simulink model "Full_Controller_SIM"  (R2026a)
settings: Solver=FixedStepDiscrete  StopTime=S.tspan  FixedStep=S.dt_sim  RelTol=rel_tol  AbsTol=abs_tol
StopFcn:
  | defaultToFileBlockNames(bdroot);
undefined symbols (not defined in the file): I, S
libraries: ros2lib x8
PreSaveFcn:
  | defaultToFileBlockNames(bdroot);
settings Model: DataDictionary=ros2lib.sldd  Creator=koryh  LastModifiedBy=kjhaydon
settings SimscapeCC: SimscapeNominalValues="[{\"value\":\"1\",\"unit\":\"A\"},{\"value\":\"1\",\"unit\":\"bar\"},{\"value\":\"1\",\"unit\":\"cm^2\"},{\"value\":\"1\",\"unit\":\"cm^3/s\"},{\"value\":\"1\",\"unit\":\"kJ/kg\"},{\"value\":\"1\",\"unit\":\"kW\"},{\"value\":\"1\",\"unit\":\"l\"},{\"value\":\"1\",\"unit\":\"N\"},{\"value\":\"1\",\"unit\":\"N*m\"},{\"value\":\"1\",\"unit\":\"V\"}]"  SimscapeLogType=none  SimscapeLogDataHistory=5000.0

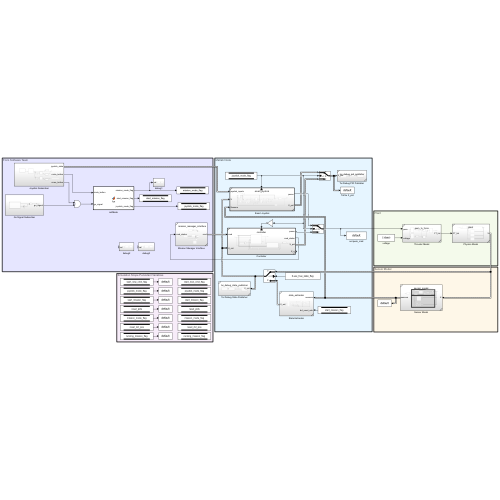
[thumbnail: Simulink's stored preview of the top-level diagram]
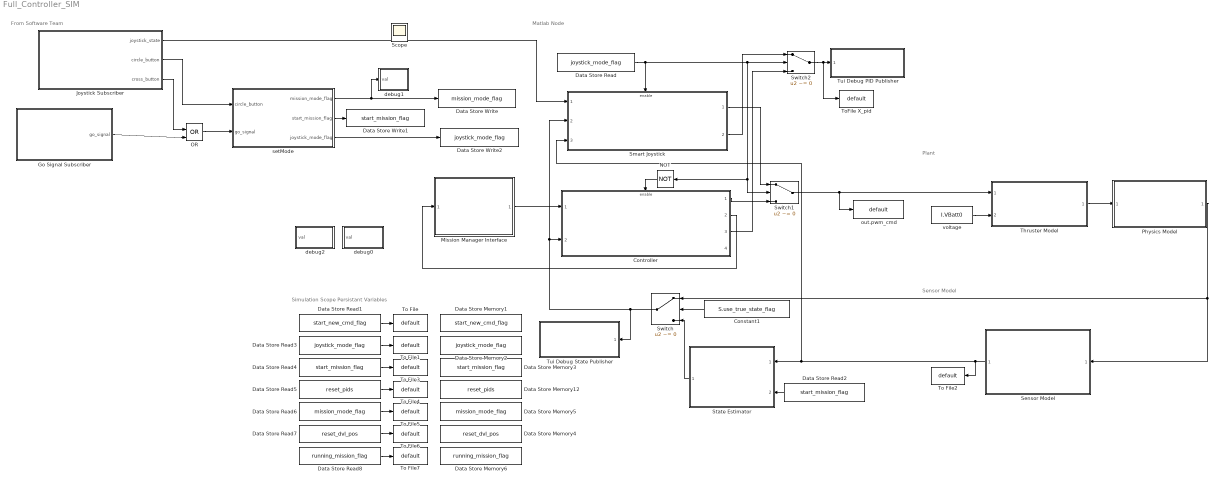
== system Full_Controller_SIM ==
  note: Sensor Model
  note: Plant
  note: Matlab Node
  note: From Software Team
  note: Simulation Scope Persistant Variables
  Constant1 : Constant  Value=S.use_true_state_flag
  Controller : Subsystem  ReferencedSubsystem=controller
  Data Store Memory1 : DataStoreMemory  DataStoreName=start_new_cmd_flag  WriteAfterWriteMsg=warning  InitialValue=true  ShowAdditionalParam=off  OutDataTypeStr=boolean
  Data Store Memory12 : DataStoreMemory  DataStoreName=reset_pids  WriteAfterWriteMsg=warning  InitialValue=false  ShowAdditionalParam=off  OutDataTypeStr=boolean
  Data Store Memory2 : DataStoreMemory  DataStoreName=joystick_mode_flag  WriteAfterWriteMsg=warning  InitialValue=S.initial_joystick_mode_enabled_flag  ShowAdditionalParam=off  OutDataTypeStr=boolean
  Data Store Memory3 : DataStoreMemory  DataStoreName=start_mission_flag  WriteAfterWriteMsg=warning  InitialValue=false  ShowAdditionalParam=off  OutDataTypeStr=boolean
  Data Store Memory4 : DataStoreMemory  DataStoreName=reset_dvl_pos  WriteAfterWriteMsg=warning  InitialValue=false  ShowAdditionalParam=off  OutDataTypeStr=boolean
  Data Store Memory5 : DataStoreMemory  DataStoreName=mission_mode_flag  WriteAfterWriteMsg=warning  InitialValue=~S.initial_joystick_mode_enabled_flag  ShowAdditionalParam=off  OutDataTypeStr=boolean
  Data Store Memory6 : DataStoreMemory  DataStoreName=running_mission_flag  WriteAfterWriteMsg=warning  InitialValue=false  ShowAdditionalParam=off  OutDataTypeStr=boolean
  Data Store Read : DataStoreRead  DataStoreName=joystick_mode_flag  IndexOptions=Index vector (dialog)  Indices=1  OutputSizes=1
  Data Store Read1 : DataStoreRead  DataStoreName=start_new_cmd_flag  IndexOptions=Index vector (dialog)  Indices=1  OutputSizes=1
  Data Store Read2 : DataStoreRead  DataStoreName=start_mission_flag  IndexOptions=Index vector (dialog)  Indices=1  OutputSizes=1
  Data Store Read3 : DataStoreRead  DataStoreName=joystick_mode_flag  IndexOptions=Index vector (dialog)  Indices=1  OutputSizes=1
  Data Store Read4 : DataStoreRead  DataStoreName=start_mission_flag  IndexOptions=Index vector (dialog)  Indices=1  OutputSizes=1
  Data Store Read5 : DataStoreRead  DataStoreName=reset_pids  IndexOptions=Index vector (dialog)  Indices=1  OutputSizes=1
  Data Store Read6 : DataStoreRead  DataStoreName=mission_mode_flag  IndexOptions=Index vector (dialog)  Indices=1  OutputSizes=1
  Data Store Read7 : DataStoreRead  DataStoreName=reset_dvl_pos  IndexOptions=Index vector (dialog)  Indices=1  OutputSizes=1
  Data Store Read8 : DataStoreRead  DataStoreName=running_mission_flag  IndexOptions=Index vector (dialog)  Indices=1  OutputSizes=1
  Data Store Write : DataStoreWrite  DataStoreName=mission_mode_flag  IndexOptions=Index vector (dialog)  Indices=1  OutputSizes=1
  Data Store Write1 : DataStoreWrite  DataStoreName=start_mission_flag  IndexOptions=Index vector (dialog)  Indices=1  OutputSizes=1
  Data Store Write2 : DataStoreWrite  DataStoreName=joystick_mode_flag  IndexOptions=Index vector (dialog)  Indices=1  OutputSizes=1
  Go Signal Subscriber : Subsystem
  Joystick Subscriber : Subsystem
  Mission Manager Interface : Subsystem  ReferencedSubsystem=mission_manager_interface
  NOT : Logic  Operator=NOT  IconShape=distinctive  AllPortsSameDT=off  OutDataTypeStr=boolean
  OR : Logic  Operator=OR  IconShape=distinctive  AllPortsSameDT=off  OutDataTypeStr=boolean
  Physics Model : Subsystem  ReferencedSubsystem=plant
  Sensor Model : Subsystem  ReferencedSubsystem=sensor_model
  Smart Joystick : Subsystem  ReferencedSubsystem=smart_joystick
  State Estimator : Subsystem  ReferencedSubsystem=state_estimator
  Switch : Switch  Criteria=u2 ~= 0  SaturateOnIntegerOverflow=off  InputSameDT=off
  Switch1 : Switch  Criteria=u2 ~= 0  SaturateOnIntegerOverflow=off  InputSameDT=off
  Switch2 : Switch  Criteria=u2 ~= 0  SaturateOnIntegerOverflow=off  InputSameDT=off
  Thruster Model : Subsystem  ReferencedSubsystem=pwm_to_force
  To File : ToFile  Filename=default  MatrixName=start_new_cmd_flag  SaveFormat=Timeseries  SampleTime=S.dt_control
  To File1 : ToFile  Filename=default  MatrixName=joystick_mode_flag  SaveFormat=Timeseries  SampleTime=S.dt_control
  To File2 : ToFile  Filename=default  MatrixName=sensors  SaveFormat=Timeseries
  To File3 : ToFile  Filename=default  MatrixName=start_mission_flag  SaveFormat=Timeseries  SampleTime=S.dt_control
  To File4 : ToFile  Filename=default  MatrixName=reset_pids  SaveFormat=Timeseries  SampleTime=S.dt_control
  To File5 : ToFile  Filename=default  MatrixName=mission_mode_flag  SaveFormat=Timeseries  SampleTime=S.dt_control
  To File6 : ToFile  Filename=default  MatrixName=reset_dvl_pos  SaveFormat=Timeseries  SampleTime=S.dt_control
  To File7 : ToFile  Filename=default  MatrixName=running_mission_flag  SaveFormat=Timeseries  SampleTime=S.dt_control
  ToFile X_pid : ToFile  Filename=default  MatrixName=X_pid  SaveFormat=Timeseries  SampleTime=S.dt_data
  Tui Debug PID Publisher : Subsystem  ReferencedSubsystem=tui_debug_pid_publisher
  Tui Debug State Publisher : Subsystem  ReferencedSubsystem=tui_debug_state_publisher
  debug0 : Subsystem
  debug1 : Subsystem
  debug2 : Subsystem
  out.pwm_cmd : ToFile  Filename=default  MatrixName=pwm_ctrl  SaveFormat=Timeseries  SampleTime=S.dt_data
  setMode : MATLAB Function  TreatAsAtomicUnit=on
  voltage : Constant  Value=I.VBatt0
  Scope : Scope
      settings: ActiveDisplayYMinimum=-0.048832566475369238  ActiveDisplayYMaximum=0.79721663606048965
  wires:
  voltage/1 -> Thruster Model/2
  Thruster Model/1 -> Physics Model/1
  Physics Model/1 -> Sensor Model/1, Switch/1
  Sensor Model/1 -> To File2/1, State Estimator/1, Smart Joystick/3
  Switch/1 -> Controller/2, Smart Joystick/2, Tui Debug State Publisher/1
  Constant1/1 -> Switch/2
  State Estimator/1 -> Switch/3
  Data Store Read2/1 -> State Estimator/2
  Controller/1 -> Switch1/3
  Switch1/1 -> out.pwm_cmd/1, Thruster Model/1
  Controller/2 -> Mission Manager Interface/1
  Go Signal Subscriber/1(go_signal) -> OR/2
  Joystick Subscriber/2(circle_button) -> setMode/1(circle_button)
  Joystick Subscriber/3(cross_button) -> OR/1
  setMode/3(joystick_mode_flag) -> Data Store Write2/1
  setMode/2(start_mission_flag) -> Data Store Write1/1
  setMode/1(mission_mode_flag) -> debug1/1(val), Data Store Write/1
  OR/1 -> setMode/2(go_signal)
  Mission Manager Interface/1 -> Controller/1
  NOT/1 -> Controller/Enable
  Data Store Read/1 -> Smart Joystick/Enable, NOT/1, Switch1/2, Switch2/2
  Smart Joystick/1 -> Switch1/1
  Joystick Subscriber/1(joystick_state) -> Smart Joystick/1
  Switch2/1 -> ToFile X_pid/1, Tui Debug PID Publisher/1
  Smart Joystick/2 -> Switch2/1
  Controller/3 -> Switch2/3
  Data Store Read3/1 -> To File1/1
  Data Store Read7/1 -> To File6/1
  Data Store Read1/1 -> To File/1
  Data Store Read5/1 -> To File4/1
  Data Store Read4/1 -> To File3/1
  Data Store Read6/1 -> To File5/1
  Data Store Read8/1 -> To File7/1

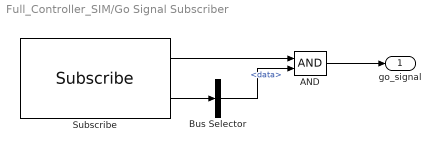
== system Full_Controller_SIM/Go Signal Subscriber ==
  AND : Logic  IconShape=distinctive  AllPortsSameDT=off  OutDataTypeStr=boolean
  Bus Selector : BusSelector  OutputSignals=data
  Subscribe : ros2lib/Subscribe  topicSource=Specify your own  topic=/go_signal  messageType=std_msgs/Bool  sampleTime=-1  QOSHistory=Keep last  QOSDepth=10  QOSReliability=Reliable  QOSDurability=Volatile  QOSDeadline=Inf  QOSLifespan=Inf  QOSLiveliness=Automatic  QOSLeaseDuration=Inf  QOSAvoidROSNamespaceConventions=off
  go_signal : Outport
  wires:
  Subscribe/2 -> Bus Selector/1
  Subscribe/1 -> AND/1
  Bus Selector/1 -> AND/2  "<data>"
  AND/1 -> go_signal/1

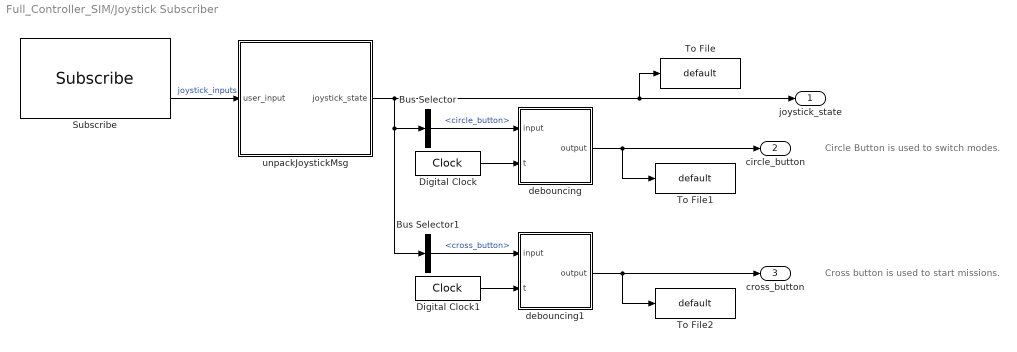
== system Full_Controller_SIM/Joystick Subscriber ==
  note: Circle Button is used to switch modes.
  note: Cross button is used to start missions.
  Bus Selector : BusSelector  OutputSignals=circle_button
  Bus Selector1 : BusSelector  OutputSignals=cross_button
  Digital Clock : DigitalClock  SampleTime=S.dt_control
  Digital Clock1 : DigitalClock  SampleTime=S.dt_control
  Subscribe : ros2lib/Subscribe  topicSource=Specify your own  topic=/ps5_controller  messageType=custom_interfaces/Gamepad  sampleTime=1/100  QOSHistory=Keep last  QOSDepth=10  QOSReliability=Reliable  QOSDurability=Volatile  QOSDeadline=Inf  QOSLifespan=Inf  QOSLiveliness=Automatic  QOSLeaseDuration=Inf  QOSAvoidROSNamespaceConventions=off
  To File : ToFile  Filename=default  MatrixName=joystick_state  SaveFormat=Timeseries  SampleTime=S.dt_control
  To File1 : ToFile  Filename=default  MatrixName=circle_button  SaveFormat=Timeseries  SampleTime=S.dt_control
  To File2 : ToFile  Filename=default  MatrixName=cross_button  SaveFormat=Timeseries  SampleTime=S.dt_control
  debouncing : MATLAB Function  TreatAsAtomicUnit=on
  debouncing1 : MATLAB Function  TreatAsAtomicUnit=on
  unpackJoystickMsg : MATLAB Function  TreatAsAtomicUnit=on
  joystick_state : Outport
  circle_button : Outport  Port=2
  cross_button : Outport  Port=3
  wires:
  Subscribe/2 -> unpackJoystickMsg/1(user_input)  "joystick_inputs"
  debouncing/1(output) -> circle_button/1, To File1/1
  Digital Clock/1 -> debouncing/2(t)
  Bus Selector/1 -> debouncing/1(input)  "<circle_button>"
  unpackJoystickMsg/1(joystick_state) -> To File/1, joystick_state/1, Bus Selector1/1, Bus Selector/1
  Bus Selector1/1 -> debouncing1/1(input)  "<cross_button>"
  debouncing1/1(output) -> cross_button/1, To File2/1
  Digital Clock1/1 -> debouncing1/2(t)

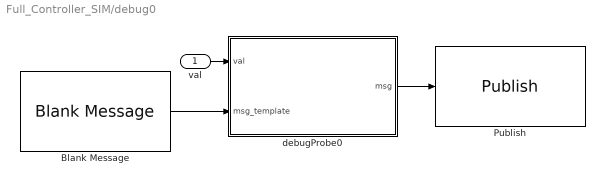
== system Full_Controller_SIM/debug0 ==
  val : Inport
  Blank Message : ros2lib/Blank Message  messageClass=Message  entityType=custom_interfaces/DebugFlag  messageType=custom_interfaces/DebugFlag  SampleTime=inf
  Publish : ros2lib/Publish  topicSource=Specify your own  topic=/matlab_debug_flag_0  messageType=custom_interfaces/DebugFlag  QOSHistory=Keep last  QOSDepth=10  QOSReliability=Reliable  QOSDurability=Volatile  QOSDeadline=Inf  QOSLifespan=Inf  QOSLiveliness=Automatic  QOSLeaseDuration=Inf  QOSAvoidROSNamespaceConventions=off
  debugProbe0 : MATLAB Function  TreatAsAtomicUnit=on
  wires:
  debugProbe0/1(msg) -> Publish/1
  val/1 -> debugProbe0/1(val)
  Blank Message/1 -> debugProbe0/2(msg_template)

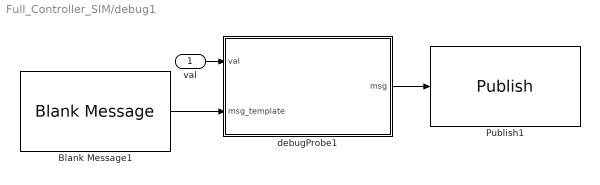
== system Full_Controller_SIM/debug1 ==
  val : Inport
  Blank Message1 : ros2lib/Blank Message  messageClass=Message  entityType=custom_interfaces/DebugFlag  messageType=custom_interfaces/DebugFlag  SampleTime=inf
  Publish1 : ros2lib/Publish  topicSource=Specify your own  topic=/matlab_debug_flag_1  messageType=custom_interfaces/DebugFlag  QOSHistory=Keep last  QOSDepth=10  QOSReliability=Reliable  QOSDurability=Volatile  QOSDeadline=Inf  QOSLifespan=Inf  QOSLiveliness=Automatic  QOSLeaseDuration=Inf  QOSAvoidROSNamespaceConventions=off
  debugProbe1 : MATLAB Function  TreatAsAtomicUnit=on
  wires:
  Blank Message1/1 -> debugProbe1/2(msg_template)
  val/1 -> debugProbe1/1(val)
  debugProbe1/1(msg) -> Publish1/1

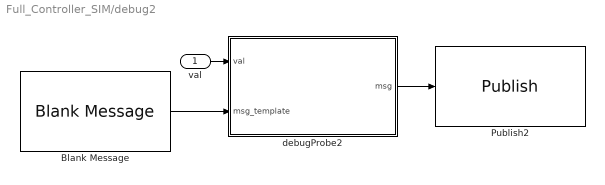
== system Full_Controller_SIM/debug2 ==
  val : Inport
  Blank Message : ros2lib/Blank Message  messageClass=Message  entityType=custom_interfaces/DebugFlag  messageType=custom_interfaces/DebugFlag  SampleTime=inf
  Publish2 : ros2lib/Publish  topicSource=Specify your own  topic=/matlab_debug_flag_2  messageType=custom_interfaces/DebugFlag  QOSHistory=Keep last  QOSDepth=10  QOSReliability=Reliable  QOSDurability=Volatile  QOSDeadline=Inf  QOSLifespan=Inf  QOSLiveliness=Automatic  QOSLeaseDuration=Inf  QOSAvoidROSNamespaceConventions=off
  debugProbe2 : MATLAB Function  TreatAsAtomicUnit=on
  wires:
  debugProbe2/1(msg) -> Publish2/1
  val/1 -> debugProbe2/1(val)
  Blank Message/1 -> debugProbe2/2(msg_template)

== matlab function Full_Controller_SIM/Joystick Subscriber/debouncing1 ==
  data: input input; output output; t input
function output  = fcn(input,t)

persistent time_of_last_pulse

if(isempty(time_of_last_pulse))
    time_of_last_pulse = t;
end


if(input)
    if(t - time_of_last_pulse <= .2)
        output = false;
    else
        output = logical(input);
    end
else
    output = false;
end

if(input)
    time_of_last_pulse = t;
end

== matlab function Full_Controller_SIM/debug0/debugProbe0 ==
  data: val input; msg output Bus: SL_Bus_custom_interfaces_DebugFlag; msg_template input Bus: SL_Bus_custom_interfaces_DebugFlag
function msg = fcn(val, msg_template)

msg = msg_template;

if(islogical(val))
    val_double = double(val);
else
    val_double = val;
end

msg.name = uint8('label___________')';
msg.value = val_double;

== matlab function Full_Controller_SIM/debug1/debugProbe1 ==
  data: val input; msg output Bus: SL_Bus_custom_interfaces_DebugFlag; msg_template input Bus: SL_Bus_custom_interfaces_DebugFlag
function msg = fcn(val, msg_template)

msg = msg_template;

if(islogical(val))
    val_double = double(val);
else
    val_double = val;
end

msg.name = uint8('miss_mode_flag__')';
msg.value = val_double;

== matlab function Full_Controller_SIM/debug2/debugProbe2 ==
  data: val input; msg output Bus: SL_Bus_custom_interfaces_DebugFlag; msg_template input Bus: SL_Bus_custom_interfaces_DebugFlag
function msg = fcn(val, msg_template)

msg = msg_template;

if(islogical(val))
    val_double = double(val);
else
    val_double = val;
end

msg.name = uint8('label___________')';
msg.value = val_double;

== matlab function Full_Controller_SIM/Joystick Subscriber/debouncing ==
  data: input input; output output; t input
function output  = fcn(input,t)

persistent time_of_last_pulse

if(isempty(time_of_last_pulse))
    time_of_last_pulse = t;
end


if(input)
    if(t - time_of_last_pulse <= .2)
        output = false;
    else
        output = logical(input);
    end
else
    output = false;
end

if(input)
    time_of_last_pulse = t;
end

== matlab function Full_Controller_SIM/Joystick Subscriber/unpackJoystickMsg ==
  data: user_input input Bus: SL_Bus_custom_interfaces_Gamepad size=[1 1]; joystick_state output Bus: joystick_bus size=[1 1]
function joystick_state  = fcn(user_input)

[joystick_state] = gamepad_parser(user_input);

== matlab function Full_Controller_SIM/setMode ==
  data: circle_button input; go_signal input; mission_mode_flag output; start_mission_flag output; joystick_mode_flag output; S parameter
function [mission_mode_flag, start_mission_flag, joystick_mode_flag] = fcn(circle_button, go_signal, S)

persistent joystick_mode_flag_ mission_mode_flag_ 

%initial conditions set in createSim.m
if(isempty(joystick_mode_flag_))
    joystick_mode_flag_ = S.initial_joystick_mode_enabled_flag;
    mission_mode_flag_ = ~joystick_mode_flag_;
end

if(circle_button) %switch modes
    joystick_mode_flag_ = ~joystick_mode_flag_;
    mission_mode_flag_ = ~joystick_mode_flag_;
end

%send start signal
if(go_signal && joystick_mode_flag_)
    joystick_mode_flag_ = false;
    mission_mode_flag_ = true;
    start_mission_flag = true;
elseif(go_signal && mission_mode_flag_)
    joystick_mode_flag_ = false;
    mission_mode_flag_ = true;
    start_mission_flag = true;
else
    start_mission_flag = false;
end


mission_mode_flag = mission_mode_flag_;
joystick_mode_flag = joystick_mode_flag_;



end
